simulink model "InvertedPendulum_SwingUpBalance_RL"  (R2025b)
settings: Solver=FixedStepAuto  StartTime=0.0  StopTime=12  FixedStep=0.02  RelTol=1e-3
model workspace (MAT data in the model file):
  Bp = 0.00017
  Fc_cart = 1.8
  Kd = 0.05
  L = 0.3365
  Vp = 100
  W_ENERGY = 1
  action_delay_steps = 0
  angle_limit_for_done = inf
  dtheta0 = 0
  dx0 = 0
  enable_coulomb_cart_friction = 1
  encoder_res = 4096
  g = 9.81
  lp = 0.1778
  mCart = 1.025
  mPend = 0.11
  noise_theta = 0.0018
  noise_thetadot = 0.213
  noise_v = 0.031
  noise_x = 0.00044
  obs_delay_steps = 0
  pinion_radius = 0.00635
  rho_coulomb = 100
  theta0 = 0
  theta_offset = 0
  thetadot0 = 0
  use_sensor_effects = 0
  vel_filter_alpha = 1
  vel_filter_tau = 0
  vel_obs_gain = 1
  voltage_bias = -0.181
  voltage_deadzone = 0.2
  voltage_rate_limit = 10000
  voltage_scale = 0.8
  x0 = 0
  x_offset = 0
  x_safe = 0.35
  xdot0 = 0
  xmax = 0.407
values from neighbouring files (symbols this model uses):
  N = start at stage N    [train_InvertedPendulum_SwingUpBalance_RL.m]
  s = num2str(Ts); set_param(mdl,'FixedStep',s)    [train_InvertedPendulum_SwingUpBalance_RL.m]
  Y = 6 .* X    [scaleToVoltage.m]
undefined symbols (not defined in the file or in its folder): dspblkCoreblockFVToolHelper, gcbh, X, Z
libraries: sm_lib x21, nesl_utility x11, fl_lib x7, ee_lib x1, sdl_lib x1, rllib x1
settings Model: SimulationMode=accelerator  Creator=Abdal  LastModifiedBy=Abdal
settings DataIOCC: SignalLogging=off
settings OptimizationCC: DefaultParameterBehavior=Inlined  LocalBlockOutputs=off
settings SFSimCC: UsePrecompiledLibraries=Avoid
settings RTWCC: SystemTargetFile=TwinCatGrt.tlc  GenCodeOnly=on  GenerateMakefile=off  TemplateMakefile=tcgrt_msbuild.tmf  TargetLang=C++  Description=TwinCAT GRT Target
settings STFCustomTargetCC: SystemTargetFile=TwinCatGrt.tlc  TargetLangStandard=C++11 (ISO)  CombineOutputUpdateFcns=on  CodeInterfacePackaging=Reusable function  CPPClassGenCompliant=on  GRTInterface=off  GenerateAllocFcn=on  TcProject_BuildWithWdk=inherit default  TcCom_ExecutionSequence=UpdateBeforeOutputMapping  TcCom_OnlineChange=off  TcProject_CreateUniqueEnumItemNames=off  TcProject_DataExchangeModulesVersion=$<ModuleGenerator:DataExchange:Version>  TcCom_OutputReadOnly=on  TcProject_UseDataExchangeModules=off  TcProject_CppLanguageStandard=Default  TcProject_UseLLVMCodeInfo=on  TcProject_UseNativeBlockDiagramExport=off  TcProject_UseCodeInfoExporter=on  TcCom_OemLicenses=$<Project:OemLicenses>  TcCom_InitExceptionHandling=CallerExceptions  TcCom_StepSizeAdaptation=RequireMatchingTaskCycleTime  TcCom_OutputDataAccess=Output Source DataArea  TcProject_PublishTcUMx86=off  TcCom_ExtModeRtAllowExecutionCommands=off  TcPlcFb_Generate=on  TcCom_BlockIoDataAccess=Internal DataArea  TcCom_AllowDataAreaForSharedData=off  TcCom_ParametersCreateSymbols=on  TcPlcFb_InitExceptionHandling=CallerExceptions  TcPlcFb_ExtModeRtWaitForStart=off  TcProject_CoderCppNamespace=coder  TcCom_DWorkCreateSymbols=on  TcProject_DeployRestart=off  TcProject_PublishConfiguration=Release  TcProject_UseIntrinsics=on  TcCom_GroupIcon=$<TE140x:Icon>  TcCom_ModuleCaller=CyclicTask  TcProject_EnableNewPlatforms=off  TcProject_SignTwinCatCertName=test  TcCom_ModuleIcon=$<TE140x:Icon>  TcCom_InputInitValues=off  TcProject_IgnorePseudoArrayDimensions=off  TcCom_GroupDisplayName=$<GroupName>  TcCom_ParametersInitValues=on  TcProject_GeneratePlcLibrary=off  TcCom_ResolveMaskedSubsystems=off  TcProject_ProductName=$<ModuleGenerator:ProductId> $<ModuleGenerator:Version:MAJOR.MINOR>  TcCom_ParametersReadOnly=off  TcCom_DWorkDataAccess=Internal DataArea  TcCom_ExecuteModelCode=on  TcProject_Generate=on  TcCom_BlockDiagramExport=on  TcProject_ClassFactoryName=$<Project:Name>  TcCom_TcComWrapperFb=off  TcProject_IncrementVersion=Revision  TcCom_VariableSymbolMapping=Identical  TcProject_PublishTcOSx64=on  TcCom_ExecutionInfoParam=on  TcPlcFb_ExtModeRtAllowExecutionCommands=off  TcProject_LibraryCategories=$<VendorName>  TcCom_MaxInternalDataAreaParts=5U  TcProject_MaxVisibleArrayElements=200U  TcCom_BlockIoReadOnly=on  TcCom_ContStateDataAccess=Internal DataArea  TcCom_BlockIoCreateSymbols=on  TcProject_PublishTcOSARMv7A=off  TcPlcFb_OemLicenses=$<Project:OemLicenses>  TcProject_VendorName=TE140x Module Vendor  TcProject_UseStaticStlString=off  TcProject_TmxInstall=on  TcProject_GenerateStructDutsWithDefaultValues=Auto  TcProject_BuildSystem=Auto  TcCom_OriginalIoBlockNames=off  TcCom_InputCreateSymbols=on  TcCom_ExtendSignalResolution=off  TcPlcFb_ExtModeRtAllowForParameterChange=off  TcCom_UpdateExceptionHandling=CallerExceptions  TcCom_ParametersDataAccess=Internal DataArea  TcCom_StrictAccessLock=on  TcProject_Publish=on  TcProject_InstallPlcLibrary=off  TcProject_PublishTcOSARMv7M=off  TcCom_MonitorExecutionTime=off  TcProject_UseTmxExtension=Auto  TcCom_ContStateReadOnly=on  TcCom_GroupName=TE140x|Simulink Modules  TcProject_CLanguageStandard=Default  TcProject_Versioning=Versioned  TcProject_PublishTcRTx64=on  TcCom_BlockDiagramVariableAccess=AssignToParent  TcPlcFb_UpdateExceptionHandling=CallerExceptions  TcCom_OutputCreateSymbols=on  TcProject_PublishTcOSARMv8A=off  TcCom_DataStoreReadOnly=off  TcProject_Description=TwinCAT executable file, generated by TwinCAT $<ModuleGenerator:ProductId>  TcCom_CallerVerification=Default  TcProject_DrvProductVersion=$<DrvFileVersion>  TcProject_LowestCompatibleTcBuild=$<TwinCAT:Version:BUILD>  TcProject_ForceRebuildForPublish=off  TcCom_ExecutionInfoOutput=off  TcProject_PreferIntOverLong=off  TcCom_DataStoreDataAccess=None  TcCom_TcComWrapperFbProperties=off  TcProject_StaticStlStringCapacity=Auto  TcCom_InputReadOnly=off  TcProject_UseCodeDescriptor=on  TcCom_TcComWrapperFbPropertyMonitoring=NoMonitoring  TcCom_AccessLockState=Auto  TcCom_DWorkReadOnly=on  TcCom_GlobalParamDefaultSharing=Define  TcProject_GenerateVsSolution=No  TcProject_Verbosity=Normal  TcCom_ContStateCreateSymbols=on  TcCom_ExtModeRtWaitForStart=off  TcProject_PublishPlatformtoolset=Auto  TcCom_Legacy_ModuleBuildInfoParam=on  TcCom_Generate=on  TcProject_PublishParallel=on  TcProject_CreateScopedEnums=Auto  TcPlcFb_MonitorExecutionTime=off  TcCom_VariableSymbolMappingCustom=$<ModelName>_U=Input|$<ModelName>_Y=Output|$<ModelName>_P=ModelParameters|$<ModelName>_B=BlockIO|$<ModelName>_DW=DWork|$<ModelName>_X=ContStates  TcCom_InputDataAccess=Input Destination DataArea  TcProject_PublishTcRTx86=on  TcProject_PlcVarPrefixes=PVOID=p | BOOL=b | BOOL32=b | DATE=d | TIME_OF_DATE=td | TIME=t | LTIME=t | GUID=n  TcCom_ExtModeRtAllowForParameterChange=off  TcProject_LibCatPath=$<Project:Dir>\$<Project:Name>.libcat.xml  TcCom_OnlineChangeRestoreDataAreas=off  TcProject_VersionSrc=$<LatestTMFile>  TcCom_BlockDiagramDebugInfoExport=on  TcProject_VendorIcon=$<TE140x:Icon>  TcProject_PublishTcUMx64=off  TcProject_SignWithTwinCatCertificate=inherit default  TcProject_Copyright=Copyright $<VendorName> $<LocalDateTime:%Y>  TcCom_DataStoreCreateSymbols=on  TcProject_DrvFileVersion=$<VersionFromFile>  TcProject_UseDescriptorCodeType=on  TcProject_PreferToolArchitectureX64=on
settings GRTTargetCC: ExtModeMexFile=TcExtModeClient  TargetLangStandard=C++11 (ISO)  ParMdlRefBuildCompliant=off  CompOptLevelCompliant=off  MatFileLogging=off  CodeInterfacePackaging=Reusable function  GenerateAllocFcn=on  UseToolchainInfoCompliant=off
settings SimscapeCC: SimscapeLogToSDI=on

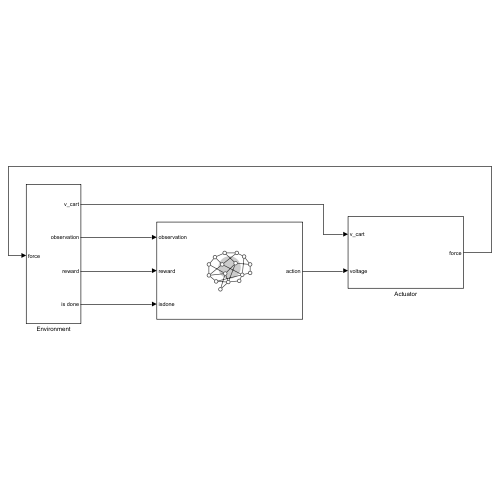
[thumbnail: Simulink's stored preview of the top-level diagram]
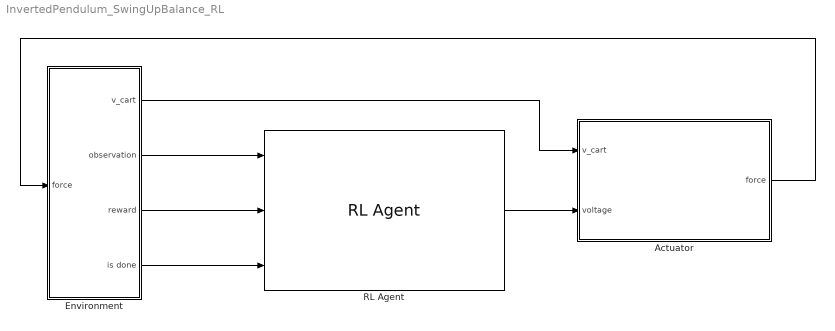
== system InvertedPendulum_SwingUpBalance_RL ==
  Actuator : Subsystem
  Environment : Subsystem
  RL Agent : rllib/RL Agent  Agent=agent  ExternalActionAsInput=off  ProvideLastAction=off  ProvideCumRwd=off  TreatAsDirectFeedthrough=on  UseStrictObservationDataTypes=off
  wires:
  Environment/1(v_cart) -> Actuator/1(v_cart)
  Actuator/1(force) -> Environment/1(force)
  Environment/2(observation) -> RL Agent/1
  Environment/4(is done) -> RL Agent/3
  Environment/3(reward) -> RL Agent/2
  RL Agent/1 -> Actuator/2(voltage)

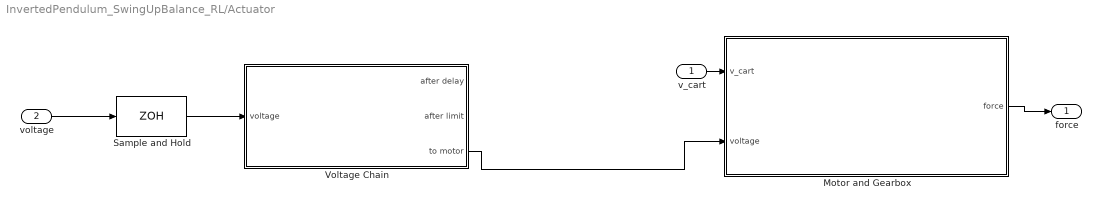
== system InvertedPendulum_SwingUpBalance_RL/Actuator ==
  v_cart : Inport
  voltage : Inport  Port=2
  Motor and Gearbox : Subsystem  Description=DC motor, gearbox and pinion. In: voltage. Out: force on the cart.
  Sample and Hold : ZeroOrderHold  SampleTime=0.02
      settings: AttributesFormatString=Ts=%<SampleTime>
  Voltage Chain : Subsystem  Description=Delay, gain, offset, rate limit, dead zone and +/-6 V limit.
  force : Outport
  wires:
  voltage/1 -> Sample and Hold/1
  Sample and Hold/1 -> Voltage Chain/1(voltage)
  Voltage Chain/3(to motor) -> Motor and Gearbox/2(voltage)
  Motor and Gearbox/1(force) -> force/1
  v_cart/1 -> Motor and Gearbox/1(v_cart)

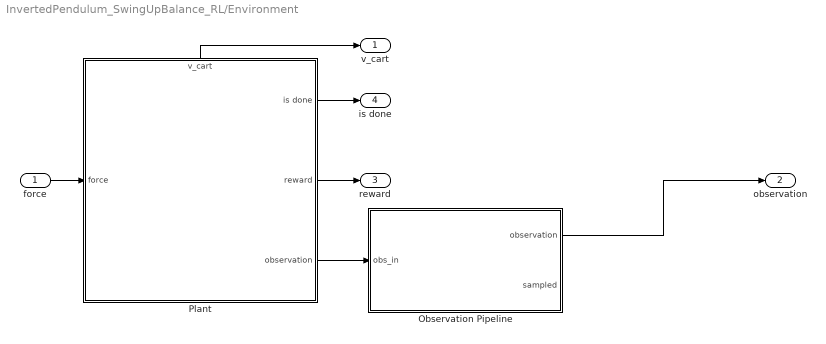
== system InvertedPendulum_SwingUpBalance_RL/Environment ==
  force : Inport
  Observation Pipeline : Subsystem
  Plant : Subsystem  Description=Cart-pole, observations and reward. Outputs: is done, reward, observation, v_cart.
      settings: PortSchema="{\"entries\":[{\"content\":{\"sides\":[{\"content\":{\"connectorIds\":[\"In1\"]},\"type\":\"ConnectorPlacement.EquallySpacedRectSide\",\"uuid\":\"3bf61207-e9a9-4acd-880c-0840df266536\"},{\"content\":{\"connectorIds\":[\"Out1\",\"Out2\",\"Out3\"],\"side\":\"RIGHT\"},\"type\":\"ConnectorPlacement.EquallySpacedRectSide\",\"uuid\":\"259f0852-313b-4e60-894f-595d7bbc28fc\"},{\"content\":{\"connectorIds\":[\"Out4\"],\"side\":\"TOP\"},\"type\":\"ConnectorPlacement.EquallySpacedRectSide\",\"uuid\":\"38486042-32ac-4db4-85e4-21220e884d32\"}]},\"type\":\"ConnectorPlacement.EquallySpacedConnector\",\"uuid\":\"6496bd53-67b6-4ee9-8103-9ef81e28ab7b\"}],\"packageUris\":[\"http://schema.mathworks.com/mf0/Connector/R2020b\"],\"version\":\"1.0\"}"
  v_cart : Outport
  observation : Outport  Port=2
  reward : Outport  Port=3
  is done : Outport  Port=4
  wires:
  Plant/3(observation) -> Observation Pipeline/1(obs_in)
  Observation Pipeline/1(observation) -> observation/1
  force/1 -> Plant/1(force)
  Plant/4(v_cart) -> v_cart/1
  Plant/1(is done) -> is done/1
  Plant/2(reward) -> reward/1

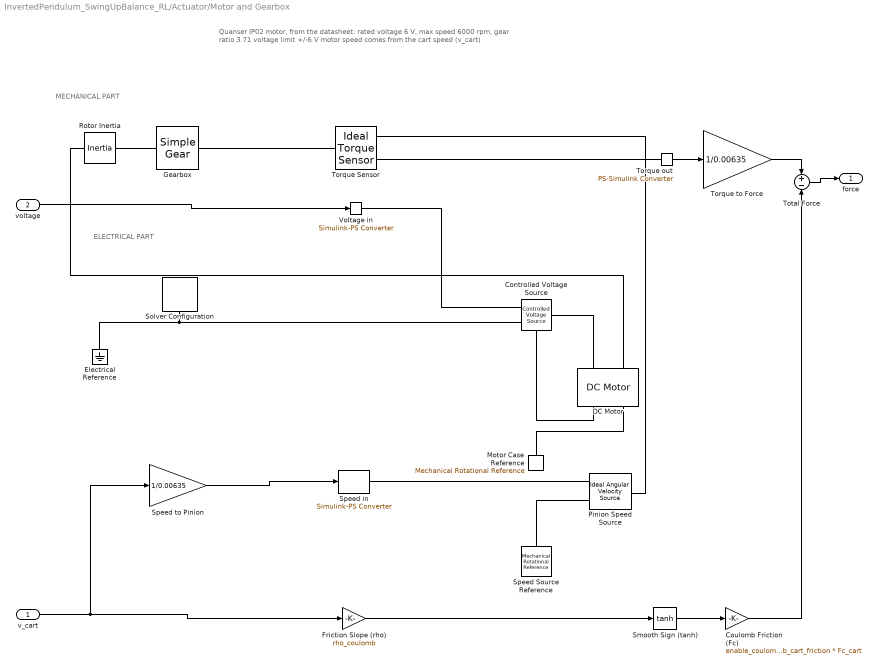
== system InvertedPendulum_SwingUpBalance_RL/Actuator/Motor and Gearbox ==
  note: Quanser IP02 motor, from the datasheet:
      | rated voltage 6 V, max speed 6000 rpm, gear ratio 3.71
      | voltage limit +/-6 V
      | motor speed comes from the cart speed (v_cart)
  note: ELECTRICAL PART
  note: MECHANICAL PART
  v_cart : Inport
  voltage : Inport  Port=2
  Controlled Voltage Source : fl_lib/Electrical/Electrical Sources/Controlled Voltage Source
  Coulomb Friction (Fc) : Gain  Gain=enable_coulomb_cart_friction * Fc_cart
  DC Motor : ee_lib/Electromechanical/Brushed Motors/DC Motor  Description=|  field_option=ee.enum.field_option.pm  Rf=100 Ohm  Lf=1 H  Laf=0.15 H  If0=0 A  parameterization=ee.enum.dcparam_option.torque_speed  Ra=2.6 Ohm  La=0.00018 H  emf_or_torque=ee.enum.emf_or_torque.ki  Kv="7.68e-3  V*s/rad"  Ki=0.818 N*m/A  T_stall="0.01709  N*m"  w_max=6000 rpm  w_rated=15000 rpm  P_rated=0.08 W  V_rated=6 V  lam_param=ee.enum.lam_param.current  i_noload=0.080 A  V_i_noload=6 V  J=0 cm^2*g  lam=0.0 N*m*s/rad  speed0=0 rpm  alpha=3.93e-3 1/K  Tmeas=25 degC  thermal_mass=100 J/K  initial_temperature=25 degC
      | Simscape DC motor. From the datasheet: 6 V rated, 6000 rpm max.
      | I could not find these values in the datasheet: rated speed 15000 rpm, Ki 0.818 N*m/A,
      | Ra 2.6 Ohm, La 0.18 mH, stall torque 17.09 mNm, rated power 0.08 W, start temperature 115 C.
  Electrical Reference : fl_lib/Electrical/Electrical Elements/Electrical Reference
  Friction Slope (rho) : Gain  Gain=rho_coulomb
  Gearbox : sdl_lib/Gears/Simple Gear  Description=Gear ratio 3.71:1  ratio=3.71  rotation_direction=sdl.enum.shaftOutputDirection.same  friction_model=sdl.enum.gear_efficiencies_load.off  T_noload=0.1 N*m  T_nom=5 N*m  efficiency_nom=0.8  efficiency=0.8  temperature_TLU=[280, 300, 320] K  load_TLU=[1, 5, 10] N*m  efficiency_TLU=[.95, .9, .85]  efficiency_TLU2=[.85, .8, .75; .95, .9, .85; .85, .8, .7]  w_thr=0.01 rad/s  pwr_thr=0.001 W  enable_backlash=false  hardstop_model=simscape.enum.hardstop.smooth  backlash_distance=1e-3 mm  r_base=0.1 m  transition=1e-4 mm  backlash_stiffness=1e6 N/m  backlash_damping=1e3 N*s/m  coeff_rest=0.7  v_tol=0.001 m/s  f_tol=0.001 N  mu_visc=[0, 0] N*m*s/rad  thermal_mass=50 J/K  temperature_specify=off  temperature_priority=None  temperature=300 K  temperature_nominal_specify=off  temperature_nominal_value=1  temperature_nominal_unit=K  x_backlash_specify=off  x_backlash_priority=None  x_backlash=0 mm  x_backlash_nominal_specify=off  x_backlash_nominal_value=1  x_backlash_nominal_unit=mm  f_hardstop_specify=off  f_hardstop_priority=None  f_hardstop=0 N  f_hardstop_nominal_specify=off  f_hardstop_nominal_value=1  f_hardstop_nominal_unit=N  v_backlash_specify=off  v_backlash_priority=None  v_backlash=0 m/s  v_backlash_nominal_specify=off  v_backlash_nominal_value=1  v_backlash_nominal_unit=m/s
  Motor Case Reference : fl_lib/Mechanical/Rotational Elements/Mechanical Rotational Reference
  Pinion Speed Source : fl_lib/Mechanical/Mechanical Sources/Ideal Angular Velocity Source
  Rotor Inertia : fl_lib/Mechanical/Rotational Elements/Inertia  Description=J = 3.9e-7 kg*m^2 (not in the datasheet).  inertia=3.9e-7 kg*m^2  num_ports=foundation.enum.numPorts2.two  w_specify=off  w_priority=None  w=0 rad/s  w_nominal_specify=off  w_nominal_value=1  w_nominal_unit=rad/s  t_specify=off  t_priority=None  t=0 N*m  t_nominal_specify=off  t_nominal_value=1  t_nominal_unit=N*m
      settings: InternalSimscapePortConfiguration="{\"Bottom\":[],\"Left\":[{\"id\":\"I\",\"label\":\"\",\"type\":\"foundation.mechanical.rotational.rotational\"}],\"Right\":[{\"id\":\"J\",\"label\":\"\",\"type\":\"foundation.mechanical.rotational.rotational\"}],\"Top\":[]}"
  Smooth Sign (tanh) : Trigonometry  Operator=tanh
  Solver Configuration : nesl_utility/Solver Configuration  PhysicalDomain=network_engine_domain  SubClassName=solver  LeftPortType=input  RightPortType=generic  Tones=[]  Harmonics=[]  SimulateNoise=off  Profile=off  UseLocalSampling=off  EnableSwitchedLinearOptims=on  FrequencyDomain=off  UseCCode=off  RelTol=0.001  AbsTol=1e-06  MinStep=1e-09  ToWorkspace=off  RevertToSquareIcSolve=off  NumHomotopyIterations=100  PhasorMode=off  PhasorModeNumHarmonics=1  ConsistencySolver=NEWTON_XTOL_AFTER_FTOL  IndexReductionMethod=DerivativeReplacement  DoDC=on  ResidualTolerance=1e-09  ConsistencyTolSource=GLOBAL  ConsistencyAbsTol=0.001  ConsistencyRelTol=0.001  ConsistencyTolFactor=0.001  UseLocalSolver=off  LocalSolverChoice=NE_BACKWARD_EULER_ADVANCER  ResolveIndetEquations=on  FunctionEvalNumThread=1  LocalSolverSampleTime=0.001  DoFixedCost=off  MaxNonlinIter=3  MaxModeIter=2  ComputeImpulses=off  ImpulseIterations=2  LinearAlgebra=auto  LinearAlgebraNumThread=0  EquationFormulation=NE_TIME_EF  DelaysMemoryBudget=1024  AutomaticFiltering=on  FilteringTimeConstant=0.001  PartitionStorageMethod=AS_NEEDED  PartitionMemoryBudget=1024  PartitionMethod=ROBUST  MultibodyUseLocalSolver=off  MultibodyLocalSolverChoice=ODE1  MultibodyLocalSolverSampleTime=0.001
  Speed Source Reference : fl_lib/Mechanical/Rotational Elements/Mechanical Rotational Reference
  Speed in : nesl_utility/Simulink-PS Converter  PhysicalDomain=network_engine_domain  SubClassName=ps_input  LeftPortType=input  RightPortType=output  PseudoPeriodic=off  Frequencies=[]  NoiseDistribution=none  NoiseParameters=[]  Unit=1  AffineConversion=off  FilteringAndDerivatives=filter  SimscapeFilterOrder=1  InputFilterTimeConstant=0.001  UdotUserProvided=0
  Speed to Pinion : Gain  Gain=1/0.00635
  Torque Sensor : fl_lib/Mechanical/Mechanical Sensors/Ideal Torque Sensor
  Torque out : nesl_utility/PS-Simulink Converter  PhysicalDomain=network_engine_domain  SubClassName=ps_output  LeftPortType=input  RightPortType=output  PseudoPeriodic=off  Frequencies=[]  VectorFormat=inherit  Unit=inherit  AffineConversion=off
  Torque to Force : Gain  Description=Force = torque / pinion radius (0.00635 m).  Gain=1/0.00635
  Total Force : Sum  Inputs=+-
  Voltage in : nesl_utility/Simulink-PS Converter  PhysicalDomain=network_engine_domain  SubClassName=ps_input  LeftPortType=input  RightPortType=output  PseudoPeriodic=off  Frequencies=[]  NoiseDistribution=none  NoiseParameters=[]  Unit=V  AffineConversion=off  FilteringAndDerivatives=provide  SimscapeFilterOrder=1  InputFilterTimeConstant=0.001  UdotUserProvided=0
  force : Outport
  wires:
  Torque out/1 -> Torque to Force/1
  v_cart/1 -> Speed to Pinion/1, Friction Slope (rho)/1
  Speed to Pinion/1 -> Speed in/1
  voltage/1 -> Voltage in/1
  Torque to Force/1 -> Total Force/1
  Friction Slope (rho)/1 -> Smooth Sign (tanh)/1
  Smooth Sign (tanh)/1 -> Coulomb Friction (Fc)/1
  Coulomb Friction (Fc)/1 -> Total Force/2
  Total Force/1 -> force/1
  connections:
  Controlled Voltage Source/LConn1 -- DC Motor/LConn1
  Torque out/LConn1 -- Torque Sensor/RConn2
  DC Motor/LConn2 -- Rotor Inertia/LConn1
  Rotor Inertia/RConn1 -- Gearbox/LConn1
  Torque Sensor/LConn1 -- Gearbox/RConn1
  DC Motor/RConn2 -- Motor Case Reference/LConn1
  Solver Configuration/RConn1 -- Controlled Voltage Source/RConn2 -- DC Motor/RConn1 -- Electrical Reference/LConn1
  Speed in/RConn1 -- Pinion Speed Source/RConn1
  Pinion Speed Source/LConn1 -- Torque Sensor/RConn1
  Pinion Speed Source/RConn2 -- Speed Source Reference/LConn1
  Voltage in/RConn1 -- Controlled Voltage Source/RConn1

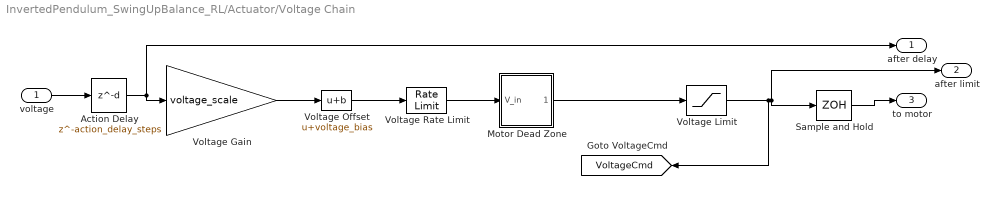
== system InvertedPendulum_SwingUpBalance_RL/Actuator/Voltage Chain ==
  voltage : Inport
  Action Delay : Delay  DelayLength=action_delay_steps  InitialCondition=0  SampleTime=0.02
  Motor Dead Zone : Subsystem
  Sample and Hold : ZeroOrderHold  SampleTime=0.02
  Voltage Gain : Gain  Gain=voltage_scale
  Voltage Limit : Saturate  UpperLimit=6  LowerLimit=-6
  Voltage Offset : Bias  Bias=voltage_bias  SaturateOnIntegerOverflow=off
  Voltage Rate Limit : RateLimiter  RisingSlewLimit=voltage_rate_limit  FallingSlewLimit=-voltage_rate_limit  SampleTimeMode=inherited
  after delay : Outport
  after limit : Outport  Port=2
  to motor : Outport  Port=3
  tag scope: VoltageCmd=global
  wires:
  voltage/1 -> Action Delay/1
  Voltage Limit/1 -> after limit/1, Sample and Hold/1, [VoltageCmd]
  Action Delay/1 -> Voltage Gain/1, after delay/1
  Sample and Hold/1 -> to motor/1
  Voltage Offset/1 -> Voltage Rate Limit/1
  Voltage Gain/1 -> Voltage Offset/1
  Voltage Rate Limit/1 -> Motor Dead Zone/1(V_in)
  Motor Dead Zone/1(V_out) -> Voltage Limit/1

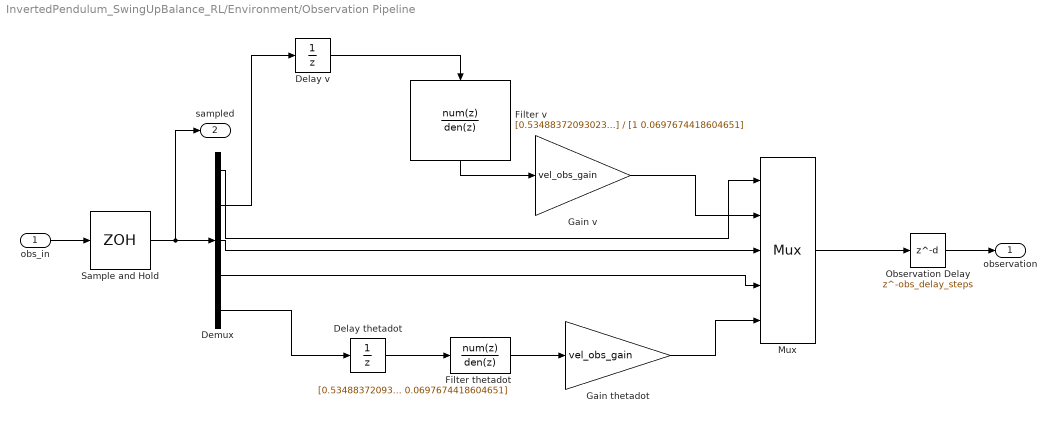
== system InvertedPendulum_SwingUpBalance_RL/Environment/Observation Pipeline ==
  obs_in : Inport
  Delay thetadot : UnitDelay  SampleTime=-1  HasFrameUpgradeWarning=on
  Delay v : UnitDelay  SampleTime=-1  HasFrameUpgradeWarning=on
  Demux : Demux  Outputs=5
  Filter thetadot : DiscreteTransferFcn  Numerator=[0.534883720930233 0.534883720930233]  Denominator=[1 0.0697674418604651]  SampleTime=0.02
  Filter v : DiscreteTransferFcn  LoadFcn=dspblkCoreblockFVToolHelper(gcbh,'load');  Numerator=[0.534883720930233 0.534883720930233]  Denominator=[1 0.0697674418604651]  SampleTime=0.02
      settings: CopyFcn=dspblkCoreblockFVToolHelper(gcbh,'copy');  DeleteFcn=dspblkCoreblockFVToolHelper(gcbh,'close');  ModelCloseFcn=dspblkCoreblockFVToolHelper(gcbh,'close');  PreSaveFcn=dspblkCoreblockFVToolHelper(gcbh,'presave');  PostSaveFcn=dspblkCoreblockFVToolHelper(gcbh,'postsave');  CloseFcn=dspblkCoreblockFVToolHelper(gcbh,'close');
  Gain thetadot : Gain  Gain=vel_obs_gain
  Gain v : Gain  Gain=vel_obs_gain
  Mux : Mux  Inputs=5
  Observation Delay : Delay  DelayLength=obs_delay_steps  InitialCondition=0  SampleTime=0.02
  Sample and Hold : ZeroOrderHold  SampleTime=0.02
  observation : Outport
  sampled : Outport  Port=2
  wires:
  obs_in/1 -> Sample and Hold/1
  Demux/2 -> Delay v/1
  Gain v/1 -> Mux/2
  Demux/5 -> Delay thetadot/1
  Demux/3 -> Mux/3
  Sample and Hold/1 -> Demux/1, sampled/1
  Demux/1 -> Mux/1
  Demux/4 -> Mux/4
  Delay v/1 -> Filter v/1
  Delay thetadot/1 -> Filter thetadot/1
  Filter v/1 -> Gain v/1
  Filter thetadot/1 -> Gain thetadot/1
  Mux/1 -> Observation Delay/1
  Gain thetadot/1 -> Mux/5
  Observation Delay/1 -> observation/1

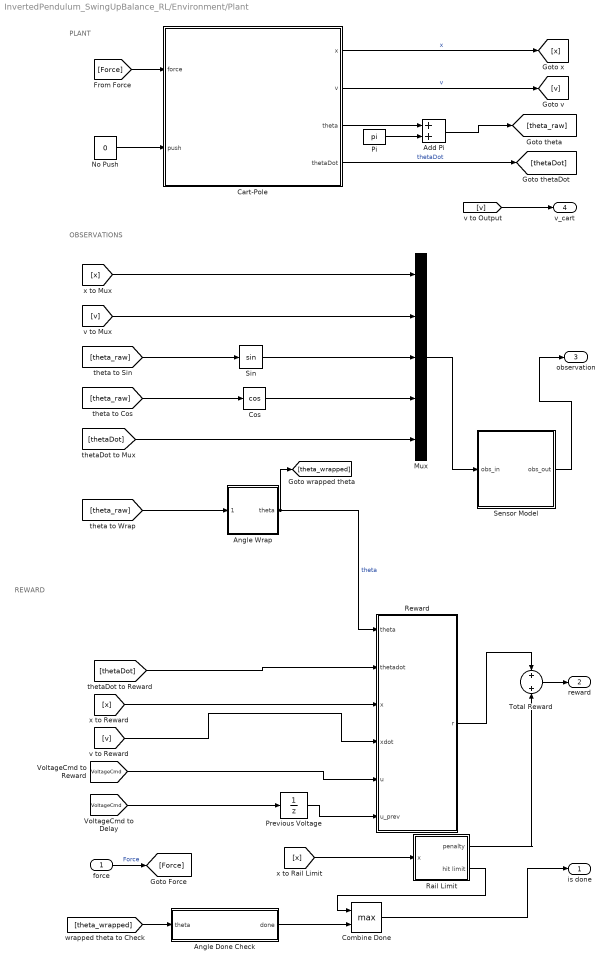
== system InvertedPendulum_SwingUpBalance_RL/Environment/Plant ==
  note: PLANT
  note: OBSERVATIONS
  note: REWARD
  force : Inport
  Add Pi : Sum
  Angle Done Check : MATLAB Function  TreatAsAtomicUnit=on
  Angle Wrap : Subsystem  Description=Keeps the angle between -pi and pi.
  Cart-Pole : Subsystem  Description=Simscape Multibody cart-pole: a sliding joint for the cart, a hinge for the pendulum.
  Combine Done : MinMax  Function=max  Inputs=2
  Cos : Trigonometry  Operator=cos
  Mux : Mux  Inputs=5
  No Push : Constant  Value=0
  Pi : Constant  Value=pi
  Previous Voltage : UnitDelay  SampleTime=-1  HasFrameUpgradeWarning=on
  Rail Limit : Subsystem  Description=Penalty and episode end when |x| > x_safe (0.35 m).
  Reward : MATLAB Function  Description=Reward: penalties, plus a bonus near the top. The training script writes new code here.  TreatAsAtomicUnit=on
  Sensor Model : MATLAB Function  TreatAsAtomicUnit=on
  Sin : Trigonometry
  Total Reward : Sum
  is done : Outport
  reward : Outport  Port=2
  observation : Outport  Port=3
  v_cart : Outport  Port=4
  wires:
  Total Reward/1 -> reward/1
  force/1 -> [Force]  "Force"
  No Push/1 -> Cart-Pole/2(push)
  [Force] -> Cart-Pole/1(force)
  [theta_raw] -> Angle Wrap/1(theta_in)
  [theta_raw] -> Cos/1
  [thetaDot] -> Mux/5
  [v] -> Mux/2
  [theta_raw] -> Sin/1
  Sin/1 -> Mux/3
  Cart-Pole/1(x) -> [x]  "x"
  Cart-Pole/2(v) -> [v]  "v"
  Cos/1 -> Mux/4
  Cart-Pole/4(thetaDot) -> [thetaDot]  "thetaDot"
  [x] -> Mux/1
  Angle Wrap/1(theta) -> Reward/1(theta), [theta_wrapped]  "theta"
  [thetaDot] -> Reward/2(thetadot)
  [x] -> Reward/3(x)
  [v] -> Reward/4(xdot)
  Previous Voltage/1 -> Reward/6(u_prev)
  [x] -> Rail Limit/1(x)
  Reward/1(r) -> Total Reward/1
  Rail Limit/1(penalty) -> Total Reward/2
  [v] -> v_cart/1
  Cart-Pole/3(theta) -> Add Pi/1
  Pi/1 -> Add Pi/2
  Add Pi/1 -> [theta_raw]
  Mux/1 -> Sensor Model/1(obs_in)
  Sensor Model/1(obs_out) -> observation/1
  [VoltageCmd] -> Reward/5(u)
  [VoltageCmd] -> Previous Voltage/1
  [theta_wrapped] -> Angle Done Check/1(theta)
  Rail Limit/2(hit limit) -> Combine Done/1
  Angle Done Check/1(done) -> Combine Done/2
  Combine Done/1 -> is done/1

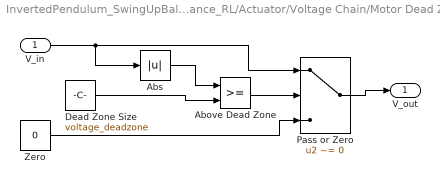
== system InvertedPendulum_SwingUpBalance_RL/Actuator/Voltage Chain/Motor Dead Zone ==
  V_in : Inport
  Above Dead Zone : RelationalOperator
  Abs : Abs
  Dead Zone Size : Constant  Value=voltage_deadzone
  Pass or Zero : Switch  Criteria=u2 ~= 0
  Zero : Constant  Value=0
  V_out : Outport
  wires:
  Abs/1 -> Above Dead Zone/1
  Dead Zone Size/1 -> Above Dead Zone/2
  Above Dead Zone/1 -> Pass or Zero/2
  Zero/1 -> Pass or Zero/3
  V_in/1 -> Abs/1, Pass or Zero/1
  Pass or Zero/1 -> V_out/1

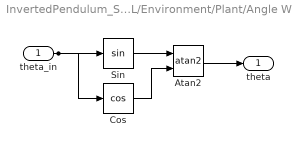
== system InvertedPendulum_SwingUpBalance_RL/Environment/Plant/Angle Wrap ==
  theta_in : Inport
  Atan2 : Trigonometry  Operator=atan2
  Cos : Trigonometry  Operator=cos
  Sin : Trigonometry
  theta : Outport
  wires:
  Atan2/1 -> theta/1
  Cos/1 -> Atan2/2
  theta_in/1 -> Cos/1, Sin/1
  Sin/1 -> Atan2/1

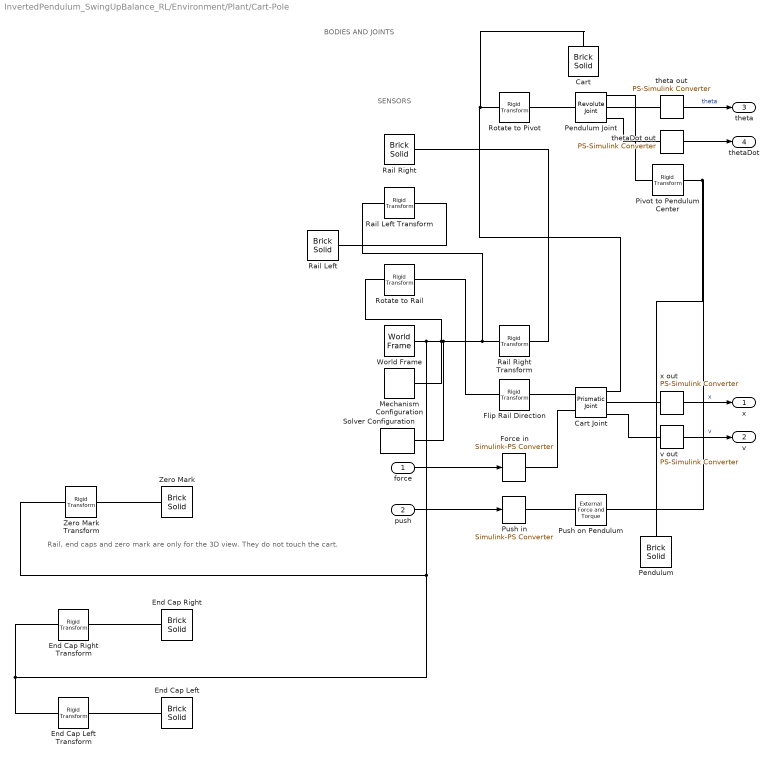
== system InvertedPendulum_SwingUpBalance_RL/Environment/Plant/Cart-Pole ==
  note: BODIES AND JOINTS
  note: SENSORS
  note: Rail, end caps and zero mark are only for the 3D view. They do not touch the cart.
  force : Inport
  push : Inport  Port=2
  Cart : sm_lib/Body Elements/Brick Solid  Description=Cart body  BrickDimensions=[0.06 0.06 0.12]  BrickDimensionsUnits=m  ExportEntireGeometry=off  InertiaType=PointMass  BasedOnType=Mass  Density=1000  DensityUnits=kg/(m^3)  Mass=mCart  MassUnits=kg  CenterOfMass=[0 0 0]  CenterOfMassUnits=m  MomentsOfInertia=[1 1 1]  MomentsOfInertiaUnits=kg*m^2  ProductsOfInertia=[0 0 0]  ProductsOfInertiaUnits=kg*m^2  GraphicType=FromGeometry  MarkerShape=Sphere  MarkerSize=10  GraphicVisPropType=SimpleVisualProperties  GraphicDiffuseColor=[0.08 0.08 0.08]  GraphicOpacity=1.0  GraphicSpecularColor=[0.5 0.5 0.5 1.0]  GraphicAmbientColor=[0.15 0.15 0.15 1.0]  GraphicEmissiveColor=[0.0 0.0 0.0 1.0]  GraphicShininess=75  DoExposeReferenceFrame=on  SerializedFrames=<Frames/>
  Cart Joint : sm_lib/Joints/Prismatic Joint  Description=Lets the cart move left and right only. The motor force acts here.  JointMode=Normal  CompositeWrenchDir=FollowerOnBase  CompositeWrenchFrame=BaseFrame  SenseConstraintForce=off  SenseConstraintTorque=off  SenseTotalForce=off  SenseTotalTorque=off  PositionTargetSpecify=on  PositionTargetPriority=High  PositionTargetValue=x0  PositionTargetValueUnits=m  VelocityTargetSpecify=on  VelocityTargetPriority=Low  VelocityTargetValue=xdot0  VelocityTargetValueUnits=m/s  EquilibriumPosition=0  EquilibriumPositionUnits=m  SpringStiffness=0  SpringStiffnessUnits=N/m  DampingCoefficient=Kd  DampingCoefficientUnits=N/(m/s)  LowerLimitSpecify=off  LowerLimitBound=2.4  LowerLimitBoundUnits=m  LowerLimitStiffness=1e6  LowerLimitStiffnessUnits=N/m  LowerLimitDamping=1e3  LowerLimitDampingUnits=N/(m/s)  LowerLimitTransitionRegionWidth=1e-4  LowerLimitTransitionRegionWidthUnits=m  UpperLimitSpecify=off  UpperLimitBound=1  UpperLimitBoundUnits=m  UpperLimitStiffness=1e6  UpperLimitStiffnessUnits=N/m  UpperLimitDamping=1e3  UpperLimitDampingUnits=N/(m/s)  UpperLimitTransitionRegionWidth=1e-4  UpperLimitTransitionRegionWidthUnits=m  TorqueActuationMode=InputTorque  MotionActuationMode=ComputedMotion  SensePosition=on  SenseVelocity=on  SenseAcceleration=off  SenseTorqueForce=off  SenseLowerLimitTorqueForce=off  SenseUpperLimitTorqueForce=off
      settings: LogSimulationData=on
  End Cap Left : sm_lib/Body Elements/Brick Solid  BrickDimensions=[0.008 0.008 0.088]  BrickDimensionsUnits=m  ExportEntireGeometry=off  InertiaType=PointMass  BasedOnType=Density  Density=1000  DensityUnits=kg/m^3  Mass=0.001  MassUnits=kg  CenterOfMass=[0 0 0]  CenterOfMassUnits=m  MomentsOfInertia=[1 1 1]  MomentsOfInertiaUnits=kg*m^2  ProductsOfInertia=[0 0 0]  ProductsOfInertiaUnits=kg*m^2  GraphicType=FromGeometry  MarkerShape=Sphere  MarkerSize=10  GraphicVisPropType=SimpleVisualProperties  GraphicDiffuseColor=[0.2 0.2 0.2]  GraphicOpacity=1  GraphicSpecularColor=[0.5 0.5 0.5 1.0]  GraphicAmbientColor=[0.15 0.15 0.15 1.0]  GraphicEmissiveColor=[0.0 0.0 0.0 1.0]  GraphicShininess=75  DoExposeReferenceFrame=on  SerializedFrames=<Frames/>
  End Cap Left Transform : sm_lib/Frames and Transforms/Rigid Transform  RotationMethod=None  FollAlignAxisA=+X  BaseAlignAxisA=+Y  FollAlignAxisB=+Y  BaseAlignAxisB=+Z  RotationStandardAxis=+Z  RotationAngle=0  RotationAngleUnits=deg  RotationArbitraryAxis=[0 0 1]  RotationSequenceAxes=FollowerAxes  RotationSequence=XYX  RotationSequenceAngles=[0 0 0]  RotationSequenceAnglesUnits=deg  RotationMatrix=[1 0 0;0 1 0;0 0 1]  Quaternion=[1 0 0 0]  TranslationMethod=Cartesian  TranslationCartesianOffset=[-0.407 0 0]  TranslationCartesianOffsetUnits=m  TranslationStandardAxis=+Z  TranslationStandardOffset=0  TranslationStandardOffsetUnits=m  TranslationROffset=0  TranslationROffsetUnits=m  TranslationThetaOffset=0  TranslationThetaOffsetUnits=deg  TranslationZOffset=0  TranslationZOffsetUnits=m
  End Cap Right : sm_lib/Body Elements/Brick Solid  BrickDimensions=[0.008 0.008 0.088]  BrickDimensionsUnits=m  ExportEntireGeometry=off  InertiaType=PointMass  BasedOnType=Density  Density=1000  DensityUnits=kg/m^3  Mass=0.001  MassUnits=kg  CenterOfMass=[0 0 0]  CenterOfMassUnits=m  MomentsOfInertia=[1 1 1]  MomentsOfInertiaUnits=kg*m^2  ProductsOfInertia=[0 0 0]  ProductsOfInertiaUnits=kg*m^2  GraphicType=FromGeometry  MarkerShape=Sphere  MarkerSize=10  GraphicVisPropType=SimpleVisualProperties  GraphicDiffuseColor=[0.2 0.2 0.2]  GraphicOpacity=1  GraphicSpecularColor=[0.5 0.5 0.5 1.0]  GraphicAmbientColor=[0.15 0.15 0.15 1.0]  GraphicEmissiveColor=[0.0 0.0 0.0 1.0]  GraphicShininess=75  DoExposeReferenceFrame=on  SerializedFrames=<Frames/>
  End Cap Right Transform : sm_lib/Frames and Transforms/Rigid Transform  RotationMethod=None  FollAlignAxisA=+X  BaseAlignAxisA=+Y  FollAlignAxisB=+Y  BaseAlignAxisB=+Z  RotationStandardAxis=+Z  RotationAngle=0  RotationAngleUnits=deg  RotationArbitraryAxis=[0 0 1]  RotationSequenceAxes=FollowerAxes  RotationSequence=XYX  RotationSequenceAngles=[0 0 0]  RotationSequenceAnglesUnits=deg  RotationMatrix=[1 0 0;0 1 0;0 0 1]  Quaternion=[1 0 0 0]  TranslationMethod=Cartesian  TranslationCartesianOffset=[0.407 0 0]  TranslationCartesianOffsetUnits=m  TranslationStandardAxis=+Z  TranslationStandardOffset=0  TranslationStandardOffsetUnits=m  TranslationROffset=0  TranslationROffsetUnits=m  TranslationThetaOffset=0  TranslationThetaOffsetUnits=deg  TranslationZOffset=0  TranslationZOffsetUnits=m
  Flip Rail Direction : sm_lib/Frames and Transforms/Rigid Transform  RotationMethod=StandardAxis  FollAlignAxisA=+X  BaseAlignAxisA=+Y  FollAlignAxisB=+Y  BaseAlignAxisB=+Z  RotationStandardAxis=+Z  RotationAngle=180  RotationAngleUnits=deg  RotationArbitraryAxis=[0 0 1]  RotationSequenceAxes=FollowerAxes  RotationSequence=XYX  RotationSequenceAngles=[0 0 0]  RotationSequenceAnglesUnits=deg  RotationMatrix=[1 0 0; 0 1 0; 0 0 1]  Quaternion=[1 0 0 0]  TranslationMethod=None  TranslationCartesianOffset=[0 0 0]  TranslationCartesianOffsetUnits=m  TranslationStandardAxis=+Z  TranslationStandardOffset=0  TranslationStandardOffsetUnits=m  TranslationROffset=0  TranslationROffsetUnits=m  TranslationThetaOffset=0  TranslationThetaOffsetUnits=deg  TranslationZOffset=0  TranslationZOffsetUnits=m
  Force in : nesl_utility/Simulink-PS Converter  PhysicalDomain=network_engine_domain  SubClassName=ps_input  LeftPortType=input  RightPortType=output  PseudoPeriodic=off  Frequencies=[]  NoiseDistribution=none  NoiseParameters=[]  Unit=1  AffineConversion=off  FilteringAndDerivatives=zero  SimscapeFilterOrder=1  InputFilterTimeConstant=0.001  UdotUserProvided=1
  Mechanism Configuration : sm_lib/Utilities/Mechanism Configuration  Description=Gravity and other settings for the mechanism.  UniformGravity=Constant  GravityVector=[0 0 -9.81]  GravityVectorUnits=m/s^2  LinearizationDelta=0.001  JointModeTransitionNonlinearIterations=2
  Pendulum : sm_lib/Body Elements/Brick Solid  Description=Pendulum rod  BrickDimensions=[L 0.01 0.01]  BrickDimensionsUnits=m  ExportEntireGeometry=off  InertiaType=CalculateFromGeometry  BasedOnType=Mass  Density=1000  DensityUnits=kg/(m^3)  Mass=mPend  MassUnits=kg  CenterOfMass=[0 0 0]  CenterOfMassUnits=m  MomentsOfInertia=[1 1 1]  MomentsOfInertiaUnits=kg*m^2  ProductsOfInertia=[0 0 0]  ProductsOfInertiaUnits=kg*m^2  GraphicType=FromGeometry  MarkerShape=Sphere  MarkerSize=10  GraphicVisPropType=SimpleVisualProperties  GraphicDiffuseColor=[0 0 1]  GraphicOpacity=1.0  GraphicSpecularColor=[0.5 0.5 0.5 1.0]  GraphicAmbientColor=[0.15 0.15 0.15 1.0]  GraphicEmissiveColor=[0.0 0.0 0.0 1.0]  GraphicShininess=75  DoExposeReferenceFrame=on  SerializedFrames=<Frames/>
  Pendulum Joint : sm_lib/Joints/Revolute Joint  Description=Lets the pendulum turn around the pivot on the cart.  JointMode=Normal  CompositeWrenchDir=FollowerOnBase  CompositeWrenchFrame=BaseFrame  SenseConstraintForce=off  SenseConstraintTorque=off  SenseTotalForce=off  SenseTotalTorque=off  PositionTargetSpecify=on  PositionTargetPriority=High  PositionTargetValue=180 + rad2deg(theta0)  PositionTargetValueUnits=deg  VelocityTargetSpecify=on  VelocityTargetPriority=Low  VelocityTargetValue=rad2deg(thetadot0)  VelocityTargetValueUnits=deg/s  EquilibriumPosition=0  EquilibriumPositionUnits=deg  SpringStiffness=0  SpringStiffnessUnits=N*m/deg  DampingCoefficient=Bp  DampingCoefficientUnits=N*m/(rad/s)  LowerLimitSpecify=off  LowerLimitBound=-90  LowerLimitBoundUnits=deg  LowerLimitStiffness=1e4  LowerLimitStiffnessUnits=N*m/deg  LowerLimitDamping=10  LowerLimitDampingUnits=N*m/(deg/s)  LowerLimitTransitionRegionWidth=0.1  LowerLimitTransitionRegionWidthUnits=deg  UpperLimitSpecify=off  UpperLimitBound=90  UpperLimitBoundUnits=deg  UpperLimitStiffness=1e4  UpperLimitStiffnessUnits=N*m/deg  UpperLimitDamping=10  UpperLimitDampingUnits=N*m/(deg/s)  UpperLimitTransitionRegionWidth=0.1  UpperLimitTransitionRegionWidthUnits=deg  TorqueActuationMode=NoTorque  MotionActuationMode=ComputedMotion  SensePosition=on  SenseVelocity=on  SenseAcceleration=off  SenseTorqueForce=off  SenseLowerLimitTorqueForce=off  SenseUpperLimitTorqueForce=off
  Pivot to Pendulum Center : sm_lib/Frames and Transforms/Rigid Transform  RotationMethod=StandardAxis  FollAlignAxisA=+X  BaseAlignAxisA=+Y  FollAlignAxisB=+Y  BaseAlignAxisB=+Z  RotationStandardAxis=+X  RotationAngle=90  RotationAngleUnits=deg  RotationArbitraryAxis=[0 0 1]  RotationSequenceAxes=FollowerAxes  RotationSequence=XYX  RotationSequenceAngles=[0 0 0]  RotationSequenceAnglesUnits=deg  RotationMatrix=[1 0 0; 0 1 0; 0 0 1]  Quaternion=[1 0 0 0]  TranslationMethod=StandardAxis  TranslationCartesianOffset=[0 0 0]  TranslationCartesianOffsetUnits=m  TranslationStandardAxis=+X  TranslationStandardOffset=lp  TranslationStandardOffsetUnits=m  TranslationROffset=0  TranslationROffsetUnits=m  TranslationThetaOffset=0  TranslationThetaOffsetUnits=deg  TranslationZOffset=0  TranslationZOffsetUnits=m
  Push in : nesl_utility/Simulink-PS Converter  PhysicalDomain=network_engine_domain  SubClassName=ps_input  LeftPortType=input  RightPortType=output  PseudoPeriodic=off  Frequencies=[]  NoiseDistribution=none  NoiseParameters=[]  Unit=1  AffineConversion=off  FilteringAndDerivatives=zero  SimscapeFilterOrder=1  InputFilterTimeConstant=0.001  UdotUserProvided=1
  Push on Pendulum : sm_lib/Forces and Torques/External Force and Torque  Description=Push on the pendulum. Input dF is 0 in training.  EnableForceX=on  EnableForceY=off  EnableForceZ=off  EnableForce=off  ForceResolutionFrame=World  EnableTorqueX=off  EnableTorqueY=off  EnableTorqueZ=off  EnableTorque=off  TorqueResolutionFrame=AttachedFrame
  Rail Left : sm_lib/Body Elements/Brick Solid  BrickDimensions=[0.814 0.008 0.008]  BrickDimensionsUnits=m  ExportEntireGeometry=off  InertiaType=PointMass  BasedOnType=Density  Density=1000  DensityUnits=kg/m^3  Mass=0.001  MassUnits=kg  CenterOfMass=[0 0 0]  CenterOfMassUnits=m  MomentsOfInertia=[1 1 1]  MomentsOfInertiaUnits=kg*m^2  ProductsOfInertia=[0 0 0]  ProductsOfInertiaUnits=kg*m^2  GraphicType=FromGeometry  MarkerShape=Sphere  MarkerSize=10  GraphicVisPropType=SimpleVisualProperties  GraphicDiffuseColor=[0.25 0.25 0.25]  GraphicOpacity=1.0  GraphicSpecularColor=[0.5 0.5 0.5 1.0]  GraphicAmbientColor=[0.15 0.15 0.15 1.0]  GraphicEmissiveColor=[0.0 0.0 0.0 1.0]  GraphicShininess=75  DoExposeReferenceFrame=on  SerializedFrames=<Frames/>
  Rail Left Transform : sm_lib/Frames and Transforms/Rigid Transform  RotationMethod=None  FollAlignAxisA=+X  BaseAlignAxisA=+Y  FollAlignAxisB=+Y  BaseAlignAxisB=+Z  RotationStandardAxis=+Z  RotationAngle=0  RotationAngleUnits=deg  RotationArbitraryAxis=[0 0 1]  RotationSequenceAxes=FollowerAxes  RotationSequence=XYX  RotationSequenceAngles=[0 0 0]  RotationSequenceAnglesUnits=deg  RotationMatrix=[1 0 0;0 1 0;0 0 1]  Quaternion=[1 0 0 0]  TranslationMethod=Cartesian  TranslationCartesianOffset=[0 0 -0.04]  TranslationCartesianOffsetUnits=m  TranslationStandardAxis=+Z  TranslationStandardOffset=0  TranslationStandardOffsetUnits=m  TranslationROffset=0  TranslationROffsetUnits=m  TranslationThetaOffset=0  TranslationThetaOffsetUnits=deg  TranslationZOffset=0  TranslationZOffsetUnits=m
  Rail Right : sm_lib/Body Elements/Brick Solid  BrickDimensions=[0.814 0.008 0.008]  BrickDimensionsUnits=m  ExportEntireGeometry=off  InertiaType=PointMass  BasedOnType=Density  Density=1000  DensityUnits=kg/m^3  Mass=0.001  MassUnits=kg  CenterOfMass=[0 0 0]  CenterOfMassUnits=m  MomentsOfInertia=[1 1 1]  MomentsOfInertiaUnits=kg*m^2  ProductsOfInertia=[0 0 0]  ProductsOfInertiaUnits=kg*m^2  GraphicType=FromGeometry  MarkerShape=Sphere  MarkerSize=10  GraphicVisPropType=SimpleVisualProperties  GraphicDiffuseColor=[0.25 0.25 0.25]  GraphicOpacity=1.0  GraphicSpecularColor=[0.5 0.5 0.5 1.0]  GraphicAmbientColor=[0.15 0.15 0.15 1.0]  GraphicEmissiveColor=[0.0 0.0 0.0 1.0]  GraphicShininess=75  DoExposeReferenceFrame=on  SerializedFrames=<Frames/>
  Rail Right Transform : sm_lib/Frames and Transforms/Rigid Transform  RotationMethod=None  FollAlignAxisA=+X  BaseAlignAxisA=+Y  FollAlignAxisB=+Y  BaseAlignAxisB=+Z  RotationStandardAxis=+Z  RotationAngle=0  RotationAngleUnits=deg  RotationArbitraryAxis=[0 0 1]  RotationSequenceAxes=FollowerAxes  RotationSequence=XYX  RotationSequenceAngles=[0 0 0]  RotationSequenceAnglesUnits=deg  RotationMatrix=[1 0 0;0 1 0;0 0 1]  Quaternion=[1 0 0 0]  TranslationMethod=Cartesian  TranslationCartesianOffset=[0 0 0.04]  TranslationCartesianOffsetUnits=m  TranslationStandardAxis=+Z  TranslationStandardOffset=0  TranslationStandardOffsetUnits=m  TranslationROffset=0  TranslationROffsetUnits=m  TranslationThetaOffset=0  TranslationThetaOffsetUnits=deg  TranslationZOffset=0  TranslationZOffsetUnits=m
  Rotate to Pivot : sm_lib/Frames and Transforms/Rigid Transform  RotationMethod=StandardAxis  FollAlignAxisA=+X  BaseAlignAxisA=+Y  FollAlignAxisB=+Y  BaseAlignAxisB=+Z  RotationStandardAxis=-X  RotationAngle=90  RotationAngleUnits=deg  RotationArbitraryAxis=[0 0 1]  RotationSequenceAxes=FollowerAxes  RotationSequence=XYX  RotationSequenceAngles=[0 0 0]  RotationSequenceAnglesUnits=deg  RotationMatrix=[1 0 0; 0 1 0; 0 0 1]  Quaternion=[1 0 0 0]  TranslationMethod=None  TranslationCartesianOffset=[0 0 0]  TranslationCartesianOffsetUnits=m  TranslationStandardAxis=+Z  TranslationStandardOffset=0  TranslationStandardOffsetUnits=m  TranslationROffset=0  TranslationROffsetUnits=m  TranslationThetaOffset=0  TranslationThetaOffsetUnits=deg  TranslationZOffset=0  TranslationZOffsetUnits=m
  Rotate to Rail : sm_lib/Frames and Transforms/Rigid Transform  RotationMethod=StandardAxis  FollAlignAxisA=+X  BaseAlignAxisA=+Y  FollAlignAxisB=+Y  BaseAlignAxisB=+Z  RotationStandardAxis=+Y  RotationAngle=90  RotationAngleUnits=deg  RotationArbitraryAxis=[0 0 1]  RotationSequenceAxes=FollowerAxes  RotationSequence=XYX  RotationSequenceAngles=[0 0 0]  RotationSequenceAnglesUnits=deg  RotationMatrix=[1 0 0; 0 1 0; 0 0 1]  Quaternion=[1 0 0 0]  TranslationMethod=None  TranslationCartesianOffset=[0 0 0]  TranslationCartesianOffsetUnits=m  TranslationStandardAxis=+Z  TranslationStandardOffset=0  TranslationStandardOffsetUnits=m  TranslationROffset=0  TranslationROffsetUnits=m  TranslationThetaOffset=0  TranslationThetaOffsetUnits=deg  TranslationZOffset=0  TranslationZOffsetUnits=m
  Solver Configuration : nesl_utility/Solver Configuration  PhysicalDomain=network_engine_domain  SubClassName=solver  LeftPortType=input  RightPortType=generic  Tones=[]  Harmonics=[]  SimulateNoise=off  Profile=off  UseLocalSampling=off  EnableSwitchedLinearOptims=on  FrequencyDomain=off  UseCCode=off  RelTol=0.001  AbsTol=1e-06  MinStep=1e-09  ToWorkspace=off  RevertToSquareIcSolve=off  NumHomotopyIterations=100  PhasorMode=off  PhasorModeNumHarmonics=1  ConsistencySolver=NEWTON_FTOL  IndexReductionMethod=DerivativeReplacement  DoDC=off  ResidualTolerance=1e-09  ConsistencyTolSource=GLOBAL  ConsistencyAbsTol=0.001  ConsistencyRelTol=0.001  ConsistencyTolFactor=0.001  UseLocalSolver=off  LocalSolverChoice=NE_BACKWARD_EULER_ADVANCER  ResolveIndetEquations=on  FunctionEvalNumThread=1  LocalSolverSampleTime=0.001  DoFixedCost=off  MaxNonlinIter=3  MaxModeIter=2  ComputeImpulses=off  ImpulseIterations=2  LinearAlgebra=Sparse  LinearAlgebraNumThread=0  EquationFormulation=NE_TIME_EF  DelaysMemoryBudget=1024  AutomaticFiltering=on  FilteringTimeConstant=0.001  PartitionStorageMethod=AS_NEEDED  PartitionMemoryBudget=1024  PartitionMethod=FAST  MultibodyUseLocalSolver=off  MultibodyLocalSolverChoice=ODE1  MultibodyLocalSolverSampleTime=0.001
  World Frame : sm_lib/Frames and Transforms/World Frame
  Zero Mark : sm_lib/Body Elements/Brick Solid  BrickDimensions=[0.005 0.005 0.025]  BrickDimensionsUnits=m  ExportEntireGeometry=off  InertiaType=PointMass  BasedOnType=Density  Density=1000  DensityUnits=kg/m^3  Mass=0.001  MassUnits=kg  CenterOfMass=[0 0 0]  CenterOfMassUnits=m  MomentsOfInertia=[1 1 1]  MomentsOfInertiaUnits=kg*m^2  ProductsOfInertia=[0 0 0]  ProductsOfInertiaUnits=kg*m^2  GraphicType=FromGeometry  MarkerShape=Sphere  MarkerSize=10  GraphicVisPropType=SimpleVisualProperties  GraphicDiffuseColor=[0.9 0.1 0.1]  GraphicOpacity=1.0  GraphicSpecularColor=[0.5 0.5 0.5 1.0]  GraphicAmbientColor=[0.15 0.15 0.15 1.0]  GraphicEmissiveColor=[0.0 0.0 0.0 1.0]  GraphicShininess=75  DoExposeReferenceFrame=on  SerializedFrames=<Frames/>
  Zero Mark Transform : sm_lib/Frames and Transforms/Rigid Transform  RotationMethod=None  FollAlignAxisA=+X  BaseAlignAxisA=+Y  FollAlignAxisB=+Y  BaseAlignAxisB=+Z  RotationStandardAxis=+Z  RotationAngle=0  RotationAngleUnits=deg  RotationArbitraryAxis=[0 0 1]  RotationSequenceAxes=FollowerAxes  RotationSequence=XYX  RotationSequenceAngles=[0 0 0]  RotationSequenceAnglesUnits=deg  RotationMatrix=[1 0 0;0 1 0;0 0 1]  Quaternion=[1 0 0 0]  TranslationMethod=Cartesian  TranslationCartesianOffset=[0 0 -0.04]  TranslationCartesianOffsetUnits=m  TranslationStandardAxis=+Z  TranslationStandardOffset=0  TranslationStandardOffsetUnits=m  TranslationROffset=0  TranslationROffsetUnits=m  TranslationThetaOffset=0  TranslationThetaOffsetUnits=deg  TranslationZOffset=0  TranslationZOffsetUnits=m
  theta out : nesl_utility/PS-Simulink Converter  PhysicalDomain=network_engine_domain  SubClassName=ps_output  LeftPortType=input  RightPortType=output  PseudoPeriodic=off  Frequencies=[]  VectorFormat=1-D array  Unit=rad  AffineConversion=off
  thetaDot out : nesl_utility/PS-Simulink Converter  PhysicalDomain=network_engine_domain  SubClassName=ps_output  LeftPortType=input  RightPortType=output  PseudoPeriodic=off  Frequencies=[]  VectorFormat=1-D array  Unit=rad/s  AffineConversion=off
  v out : nesl_utility/PS-Simulink Converter  PhysicalDomain=network_engine_domain  SubClassName=ps_output  LeftPortType=input  RightPortType=output  PseudoPeriodic=off  Frequencies=[]  VectorFormat=1-D array  Unit=m/s  AffineConversion=off
  x out : nesl_utility/PS-Simulink Converter  PhysicalDomain=network_engine_domain  SubClassName=ps_output  LeftPortType=input  RightPortType=output  PseudoPeriodic=off  Frequencies=[]  VectorFormat=1-D array  Unit=inherit  AffineConversion=off
  x : Outport  VectorParamsAs1DForOutWhenUnconnected=off
  v : Outport  Port=2  VectorParamsAs1DForOutWhenUnconnected=off
  theta : Outport  Port=3  VectorParamsAs1DForOutWhenUnconnected=off
  thetaDot : Outport  Port=4  VectorParamsAs1DForOutWhenUnconnected=off
  wires:
  force/1 -> Force in/1
  push/1 -> Push in/1
  x out/1 -> x/1  "x"
  theta out/1 -> theta/1  "theta"
  thetaDot out/1 -> thetaDot/1
  v out/1 -> v/1  "v"
  connections:
  Rail Left Transform/RConn1 -- Rail Left/RConn1
  Flip Rail Direction/RConn1 -- Cart Joint/LConn1
  Rotate to Rail/RConn1 -- Flip Rail Direction/LConn1
  Rotate to Pivot/LConn1 -- Cart Joint/RConn1 -- Cart/RConn1
  Rotate to Pivot/RConn1 -- Pendulum Joint/LConn1
  Rail Right Transform/LConn1 -- Mechanism Configuration/RConn1 -- Rotate to Rail/LConn1 -- End Cap Left Transform/LConn1 -- End Cap Right Transform/LConn1 -- Zero Mark Transform/LConn1 -- World Frame/RConn1 -- Solver Configuration/RConn1 -- Rail Left Transform/LConn1
  Rail Right Transform/RConn1 -- Rail Right/RConn1
  Push in/RConn1 -- Push on Pendulum/LConn1
  Force in/RConn1 -- Cart Joint/LConn2
  Cart Joint/RConn3 -- v out/LConn1
  Pendulum Joint/RConn1 -- Pivot to Pendulum Center/LConn1
  Pendulum Joint/RConn3 -- thetaDot out/LConn1
  Pendulum Joint/RConn2 -- theta out/LConn1
  Cart Joint/RConn2 -- x out/LConn1
  Push on Pendulum/RConn1 -- Pivot to Pendulum Center/RConn1 -- Pendulum/RConn1
  End Cap Left Transform/RConn1 -- End Cap Left/RConn1
  End Cap Right Transform/RConn1 -- End Cap Right/RConn1
  Zero Mark Transform/RConn1 -- Zero Mark/RConn1

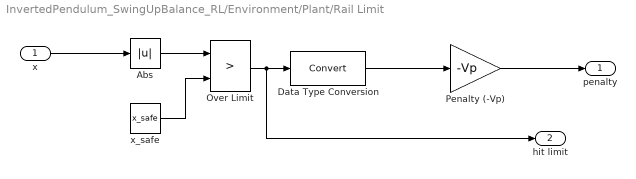
== system InvertedPendulum_SwingUpBalance_RL/Environment/Plant/Rail Limit ==
  x : Inport
  Abs : Abs  SaturateOnIntegerOverflow=off
  Data Type Conversion : DataTypeConversion  SaturateOnIntegerOverflow=off  RndMeth=Floor
  Over Limit : RelationalOperator  Operator=>  OutDataTypeStr=boolean  RndMeth=Simplest  InputSameDT=off
  Penalty (-Vp) : Gain  Gain=-Vp
  x_safe : Constant  Value=x_safe
  penalty : Outport
  hit limit : Outport  Port=2
  wires:
  x/1 -> Abs/1
  Abs/1 -> Over Limit/1
  x_safe/1 -> Over Limit/2
  Over Limit/1 -> hit limit/1, Data Type Conversion/1
  Data Type Conversion/1 -> Penalty (-Vp)/1
  Penalty (-Vp)/1 -> penalty/1

== matlab function InvertedPendulum_SwingUpBalance_RL/Environment/Plant/Sensor Model ==
  settings: updateMethod=DISCRETE  sampleTime=0.02
  data: obs_in input size=5; obs_out output size=5; use_sensor_effects parameter; encoder_res parameter; theta_offset parameter; x_offset parameter; noise_x parameter; noise_theta parameter; noise_v parameter; noise_thetadot parameter; pinion_radius parameter
function obs_out = sensor_model(obs_in, use_sensor_effects, encoder_res, theta_offset, x_offset, noise_x, noise_theta, noise_v, noise_thetadot, pinion_radius)
% adds encoder steps, offsets and noise

x_raw       = obs_in(1);
xdot_raw    = obs_in(2);
sinth_raw   = obs_in(3);
costh_raw   = obs_in(4);
thdot_raw   = obs_in(5);

if use_sensor_effects == 0
    obs_out = obs_in;
    return;
end

theta_raw = atan2(sinth_raw, costh_raw);

% encoder steps
q_theta = 2*pi / encoder_res;
theta_q = round(theta_raw / q_theta) * q_theta;
q_x = 2*pi * pinion_radius / encoder_res;
x_q = round(x_raw / q_x) * q_x;

% offsets
theta_m = theta_q + theta_offset;
x_m     = x_q + x_offset;

% noise
if noise_x > 0
    x_m = x_m + noise_x * randn();
end
if noise_theta > 0
    theta_m = theta_m + noise_theta * randn();
end

xdot_m  = xdot_raw;
thdot_m = thdot_raw;
if noise_v > 0
    xdot_m = xdot_m + noise_v * randn();
end
if noise_thetadot > 0
    thdot_m = thdot_m + noise_thetadot * randn();
end

obs_out = [x_m; xdot_m; sin(theta_m); cos(theta_m); thdot_m];
end

== matlab function InvertedPendulum_SwingUpBalance_RL/Environment/Plant/Reward ==
  data: theta input; thetadot input; x input; xdot input; u input; r output; u_prev input; W_ENERGY parameter
function r = reward_fcn(theta, thetadot, x, xdot, u, u_prev, W_ENERGY)
OMEGA_MAX = 10.0; X_MAX = 0.407; V_MAX = 1.5; U_MAX = 6.0;
W_THETA = 3.0; W_U = 0.01; W_RAIL = 15.0;
SIGMA_THETA = 0.15; SIGMA_XDOT = 0.30;
cos_th = cos(theta);
upright_blend = max(0, min(1, (-cos_th - 0.5) / 0.5));
W_X = upright_blend * 10.0000;
W_XDOT = upright_blend * 1.5000;
W_THETADOT = upright_blend * 0.1500;
W_DU = 0.02 + upright_blend * 0.2800;
BONUS = 1.0 + upright_blend * 1.0000;
SIGMA_X = 0.05 - upright_blend * 0.0150;
c_theta = (1 + cos_th) / 2;
c_thetadot = (thetadot / OMEGA_MAX)^2;
c_x = (x / X_MAX)^2;
c_xdot = (xdot / V_MAX)^2;
c_u = (u / U_MAX)^2;
c_du = ((u - u_prev) / U_MAX)^2;
RAIL_SOFT = 0.30;
x_abs = abs(x);
if x_abs > RAIL_SOFT
    c_rail = ((x_abs - RAIL_SOFT) / (X_MAX - RAIL_SOFT))^2;
else
    c_rail = 0;
end
theta_err = atan2(sin(theta - pi), cos(theta - pi));
goal_err_sq = (theta_err / SIGMA_THETA)^2 + (x / SIGMA_X)^2 + (xdot / SIGMA_XDOT)^2;
b = BONUS * exp(-0.5 * goal_err_sq);
if W_ENERGY > 0
    E_pe = (1 - cos(theta)) / 2;
    E_ke = 0.5 * (thetadot / OMEGA_MAX)^2;
    E_norm = E_pe + E_ke;
    r_energy = -W_ENERGY * (1.0 - E_norm)^2;
else
    r_energy = 0;
end
r = -W_THETA*c_theta - W_THETADOT*c_thetadot - W_X*c_x - W_XDOT*c_xdot - W_U*c_u - W_DU*c_du - W_RAIL*c_rail + b + r_energy;
end

== matlab function InvertedPendulum_SwingUpBalance_RL/Environment/Plant/Angle Done Check ==
  settings: updateMethod=DISCRETE  sampleTime=0.02
  data: theta input; done output; angle_limit_for_done parameter
function done = angle_done_fcn(theta, angle_limit_for_done)
% done when the pendulum is too far from upright (inf = off)
d = abs(atan2(sin(theta - pi), cos(theta - pi)));
if angle_limit_for_done < pi
    done = d > angle_limit_for_done;
else
    done = false;
end
end
